simulink model "dcpos_ol"  (Simulink 6.6)
settings: Solver=FixedStepDiscrete  StartTime=0.0  StopTime=inf  FixedStep=.0001  RelTol=1e-3
libraries: dsPICdrivers x7
settings Model: Creator=Kavitha  LastModifiedBy=Kavitha  ProdHWDeviceType=16-bit Generic
settings OptimizationCC: OptimizeModelRefInitCode=on  LifeSpan=1
settings HardwareCC: ProdBitPerInt=16  ProdEndianess=LittleEndian  ProdWordSize=16  ProdHWDeviceType=16-bit Generic  TargetHWDeviceType=32-bit Generic
settings RTWCC: SystemTargetFile=dspic.tlc  TemplateMakefile=dspic_pic30_gcc.tmf  PostCodeGenCommand=dsPIC_Compile()  Description=Embedded Target for Microchip dsPIC (real-time)  ProcessScript=dspic_make_rtw_hook
settings CodeAppCC: IgnoreCustomStorageClasses=off
settings STFCustomTargetCC: TargetFcnLib=ansi_tfl_tmw.mat  GenFloatMathFcnCalls=ANSI_C  ModelReferenceCompliant=off  IncludeMdlTerminateFcn=off  CombineOutputUpdateFcns=on  SuppressErrorStatus=on  ERTCustomFileBanners=on  SupportContinuousTime=off  SupportNonInlinedSFcns=off  SystemTargetFile=dspic.tlc
settings ERTTargetCC: TargetFcnLib=ansi_tfl_tmw.mat  GenFloatMathFcnCalls=ANSI_C  ModelReferenceCompliant=off  IncludeMdlTerminateFcn=off  SuppressErrorStatus=on  ModelStepFunctionPrototypeControlCompliant=off  InlinedParameterPlacement=NonHierarchical  ERTSrcFileBannerTemplate=dsPIC_code_template.cgt  ERTHdrFileBannerTemplate=dsPIC_code_template.cgt  ERTDataSrcFileTemplate=dsPIC_code_template.cgt  ERTDataHdrFileTemplate=dsPIC_code_template.cgt  ERTCustomFileTemplate=dsPIC_main.tlc
settings CustomProperty: DataType=string  Value=E:\MATLAB~1\R2007a\rtw\bin\win32\gmake

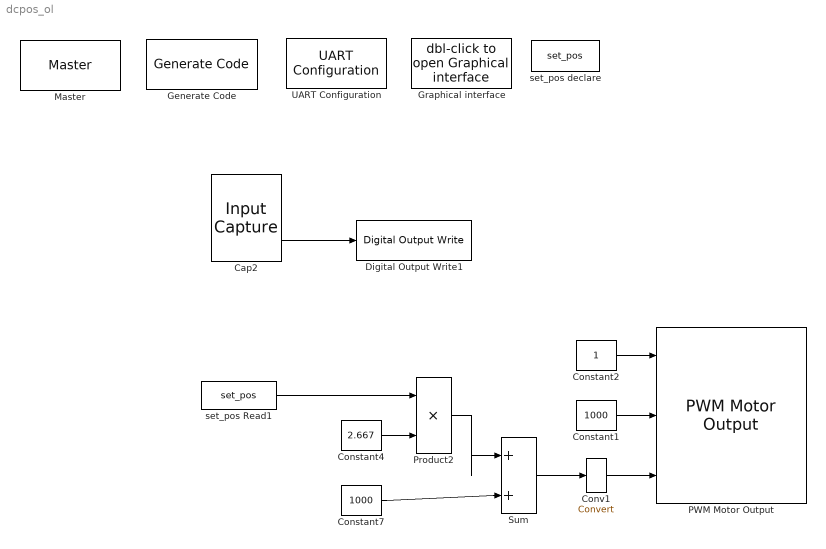
== system dcpos_ol ==
  Cap2 : dsPICdrivers/Peripheral I//O/Input Capture  Tag=dsPIC_PWM_IC  Priority=5  IntPriority=7  Channel=[7]  Channel_UP_Down_Periode=[4]  MaxChannel=[0.001]  SafeMarge=[10]  MaxName=' IC7max '  Precision=[14.4251]  Timer=[2]  ChangeDetected=[1]  ChangeDetectedPortRef=3  SampleTime=-1  Status=Channel not available on selected target
  Constant1 : Constant  Value=1000  OutDataTypeMode=uint16  SampleTime=-1
  Constant2 : Constant  OutDataTypeMode=boolean  SampleTime=-1
  Constant4 : Constant  Value=2.667  OutDataTypeMode=uint16  SampleTime=-1
  Constant7 : Constant  Value=1000  OutDataTypeMode=uint16  SampleTime=-1
  Conv1 : DataTypeConversion
  Digital Output Write1 : dsPICdrivers/Digital I//O/Digital Output Write  Tag=dsPIC_Digital_Output  Priority=5  PORT=E  Pin=[4]  Simultaneous=off  OrderingInOutPopup=None
  Generate Code : dsPICdrivers/Simulink Configuration/Generate Code
  Graphical interface : dsPICdrivers/Serial PORT/dbl-click to open Graphical interface  SystemSampleTime=-1  Nothing=0
  Master : dsPICdrivers/Master  Tag=dsPIC_MASTER  Priority=1  TimeStepType=Timer1  picType=30f4011  fcy=20e6  Quartz_33f=5e6  PLLActive_33f=off  fcyDesired_33f=0  tmr1="[1  1999  0]"  tmr1Info="Time Step : 0.0001  ;   Error : 0%  PR1=1999"  tmr2345="[1  0  0  0]"  tmr2345cfg=[-1 -1 -1 -1]  IOautoConf=on  typePort="[ 0   0   0   0   0   0   0   0   0   0   0   0   0   0   0   0   0   0   0   0   0   0   0   0   0   0   0   0   0   0   0   0   0   0   0   0   0   0   0   0   0   0   0   0   0   0   4   0   6   0   0   0   0   0   0   0   0   0   0   0   0   0   0   0   0   0   0   0  10   0   0   0   0   0   0   0   0   0   0   0   0   0   0   0   0   0   0   0   0   0   0   0   0   0   0   0   0   0   0   0   0   0   0   0   0   0   0   0   0   0   0   0 ]"  TRIS="[ 65535  65535  65535  65535  65519  65535  65535 ]"  ADPCFG=0  MasterBusyPort=None  MasterOverloadPort=None  FOSC=XT_PLL8  ClockSwitchMonitor=Both disabled  TempProtection_33f=TEMP_ON  FPBOR=PBOR_OFF  PWRT=PWRT_OFF  MCLR=MCLR_EN  PowerSave=off  OverrideFcy=off  NewFcy=1e6  PR2345="[65535  65535  65535  65535]"
  PWM Motor Output : dsPICdrivers/Peripheral I//O/PWM Motor Output  Tag=dsPIC_PWM_Motor  Priority=5  PWMref=1  PWM12=1  InputEnableChk=on  InputPeriodeChk=on  Channel=[1]  TPeriode=10e-5  PrescalerValue=1  PeriodeInteger=2000  MaxName='PWM'  Centered=off  HChannelON=on  Info="Nbr Bits : 11.9658  ||  PWM = 4000  ||  Prescaler = 1"  Delay=0  IntPriority=5  nbrPwmChannelPIC=3  Status=OK  DeadTimePrescaleA=0  DeadTimePrescaleB=0  DeadTimeInfo=Dead Time A = 0  DTPWM1a=Prescaler A  DTPWM1i=Prescaler A  DTPWM2a=Prescaler A  DTPWM2i=Prescaler A  DTPWM3a=Prescaler A  DTPWM3i=Prescaler A  DTPWM4a=Prescaler A  DTPWM4i=Prescaler A  DTCON1=0  DTCON2=0
  Product2 : Product  OutDataTypeMode=uint16  RndMeth=Zero
  Sum : Sum  Inputs=|++  OutDataTypeMode=double
  UART Configuration : dsPICdrivers/Serial PORT/UART Configuration  Tag=dsPIC_config_UART  Priority=2  UART=1  proposed_BAUD=9600  ALT_TX_RX=on  InterruptTxWhen=When Transmit Buffer is empty  TXInterruptPri=7  TxBufferSize=32  TXEN=off  InterruptRxWhen=When a character is received  RXInterruptPri=2  RxBufferSize=32  BAUD=9600  UxBRG=129  Info="UxBRG = 129   ||  Real Baud : 9615   ||  % error : 0.16026  ||  max 0.096154 Bytes / Step"  RealBaud=0
  set_pos Read1 : DataStoreRead  DataStoreName=set_pos  SampleTime=-1
  set_pos declare : DataStoreMemory  DataStoreName=set_pos  ReadBeforeWriteMsg=warning  WriteAfterWriteMsg=warning  WriteAfterReadMsg=warning  InitialValue=200  VectorParams1D=off  DataType=uint16
  wires:
  Constant2/1 -> PWM Motor Output/1
  Constant1/1 -> PWM Motor Output/2
  Constant7/1 -> Sum/2
  Sum/1 -> Conv1/1
  Conv1/1 -> PWM Motor Output/3
  Product2/1 -> Sum/1
  Constant4/1 -> Product2/2
  set_pos Read1/1 -> Product2/1
  Cap2/2 -> Digital Output Write1/1
